simulink model "MrasObserver"  (R2026b)
settings: Solver=VariableStepAuto
undefined symbols (not defined in the file or in its folder): mras_parameters
settings Model: Creator=24322  LastModifiedBy=24322

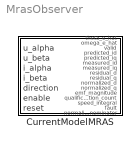
== system MrasObserver ==
  CurrentModelMRAS : Subsystem  mask{cfg=mras_parameters()}
      mask prompts: cfg "MRAS configuration"

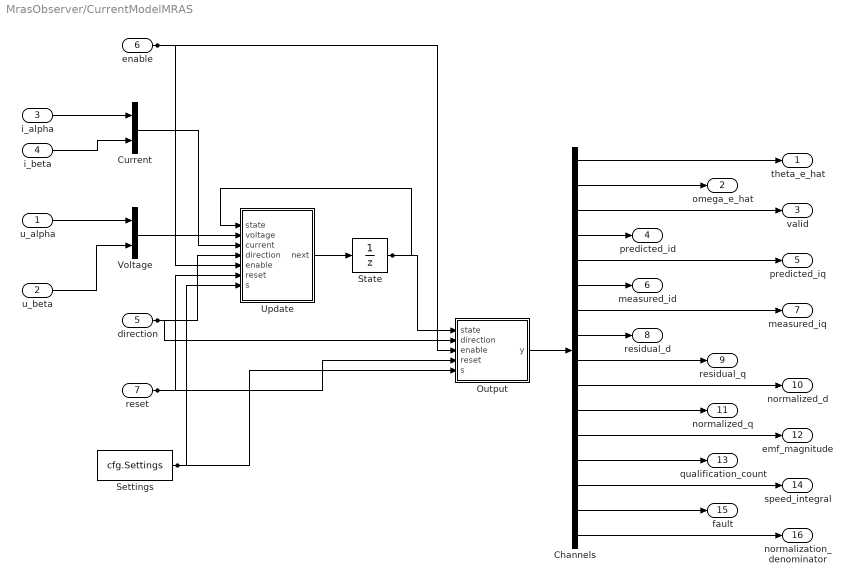
== system MrasObserver/CurrentModelMRAS ==
  u_alpha : Inport  SampleTime=cfg.Ts
  u_beta : Inport  Port=2  SampleTime=cfg.Ts
  i_alpha : Inport  Port=3  SampleTime=cfg.Ts
  i_beta : Inport  Port=4  SampleTime=cfg.Ts
  direction : Inport  Port=5  SampleTime=cfg.Ts
  enable : Inport  Port=6  SampleTime=cfg.Ts
  reset : Inport  Port=7  SampleTime=cfg.Ts
  Channels : Demux  Outputs=16
  Current : Mux  Inputs=2
  Output : MATLAB Function  TreatAsAtomicUnit=on
  Settings : Constant  Value=cfg.Settings
  State : UnitDelay  InitialCondition=zeros(21,1)  SampleTime=cfg.Ts
  Update : MATLAB Function  TreatAsAtomicUnit=on
  Voltage : Mux  Inputs=2
  theta_e_hat : Outport
  omega_e_hat : Outport  Port=2
  valid : Outport  Port=3
  predicted_id : Outport  Port=4
  predicted_iq : Outport  Port=5
  measured_id : Outport  Port=6
  measured_iq : Outport  Port=7
  residual_d : Outport  Port=8
  residual_q : Outport  Port=9
  normalized_d : Outport  Port=10
  normalized_q : Outport  Port=11
  emf_magnitude : Outport  Port=12
  qualification_count : Outport  Port=13
  speed_integral : Outport  Port=14
  fault : Outport  Port=15
  normalization_denominator : Outport  Port=16
  wires:
  Channels/16 -> normalization_denominator/1
  Channels/15 -> fault/1
  Channels/14 -> speed_integral/1
  Channels/13 -> qualification_count/1
  Channels/12 -> emf_magnitude/1
  Channels/11 -> normalized_q/1
  Channels/10 -> normalized_d/1
  Channels/9 -> residual_q/1
  Channels/8 -> residual_d/1
  Channels/7 -> measured_iq/1
  Channels/6 -> measured_id/1
  Channels/5 -> predicted_iq/1
  Channels/4 -> predicted_id/1
  Channels/3 -> valid/1
  Channels/2 -> omega_e_hat/1
  Channels/1 -> theta_e_hat/1
  Output/1(y) -> Channels/1
  Update/1(next) -> State/1
  Settings/1 -> Update/7(s), Output/5(s)
  reset/1 -> Update/6(reset), Output/4(reset)
  enable/1 -> Update/5(enable), Output/3(enable)
  direction/1 -> Update/4(direction), Output/2(direction)
  Current/1 -> Update/3(current)
  Voltage/1 -> Update/2(voltage)
  State/1 -> Update/1(state), Output/1(state)
  i_beta/1 -> Current/2
  i_alpha/1 -> Current/1
  u_beta/1 -> Voltage/2
  u_alpha/1 -> Voltage/1

== matlab function MrasObserver/CurrentModelMRAS/Output ==
  data: state input; y output; direction input; enable input; reset input; s input
function y=mras_output(state,direction,enable,reset,s)
%MRAS_OUTPUT State-only observer outputs; voltage is consumed by next-state only.
% Diagnostics describe the previous processed measurement (one Ts old).
%#codegen
y=zeros(16,1,'like',state);
if ~all(isfinite(s)) || s(1)<=0 || s(3)<=0 || s(4)<=0 || ...
        ~isfinite(enable) || ~isfinite(reset) || ~isfinite(direction) || ...
        (direction~=0 && abs(direction)~=1)
    y(15)=2;return;
end
y(1)=s(9);
if enable<.5 || reset>.5 || direction==0 || direction~=state(12),return;end
y(1)=state(1);y(2)=state(3);
y(3)=double(state(11)>=s(17) && state(20)==0);
y(4:5)=state(13:14);y(6:7)=state(4:5);y(8:9)=state(15:16);
y(10:11)=state(17:18);y(12)=state(19);y(13)=state(11);
y(14)=state(2);y(15)=state(20);y(16)=state(21);
end

== matlab function MrasObserver/CurrentModelMRAS/Update ==
  data: state input; next output; voltage input; current input; direction input; enable input; reset input; s input
function next=mras_step(state,voltage,current,direction,enable,reset,s)
%MRAS_STEP One-step measured-current model and PI speed adaptation (SPMSM).
% State and settings indices are documented in parameter/README.md.
% No integrated current estimate replaces the previous measured dq current.
%#codegen
next=state;
if isfinite(enable) && isfinite(reset) && (enable<.5 || reset>.5)
    next=zeros(21,1,'like',state);next(1)=s(9);return;
end
if ~all(isfinite(s)) || s(1)<=0 || s(3)<=0 || s(4)<=0 || ...
        ~isfinite(enable) || ~isfinite(reset) || ~isfinite(direction) || ...
        (direction~=0 && abs(direction)~=1)
    next=zeros(21,1,'like',state);next(20)=2;return;
end
if direction==0
    next=zeros(21,1,'like',state);next(1)=s(9);return;
end
if state(20)>0,next(11)=0;next(3)=0;return;end
if ~all(isfinite(voltage)) || ~all(isfinite(current))
    next(20)=1;next(11)=0;next(3)=0;return;
end
if state(12)~=direction
    next=zeros(21,1,'like',state);next(1)=s(9);
    next(2)=direction*s(10);next(3)=direction*s(10);next(12)=direction;return;
end
ts=s(1);resistance=s(2);inductance=s(3);flux=s(4);
theta=state(1);cosine=cos(theta);sine=sin(theta);
measured=[cosine*current(1)+sine*current(2);-sine*current(1)+cosine*current(2)];
applied=[cosine*voltage(1)+sine*voltage(2);-sine*voltage(1)+cosine*voltage(2)];
omega=state(3);integral=state(2);count=cast(0,'like',state);
if state(8)>.5
    previous=state(4:5);previousVoltage=state(6:7);
    predicted=previous+(ts/inductance)*(previousVoltage-resistance*previous+ ...
        omega*inductance*[previous(2);-previous(1)]-[0;omega*flux]);
    residual=measured-predicted;
    filtered=state(9:10)+s(8)*(residual-state(9:10));
    denominator=ts*omega*flux/inductance;
    floorValue=ts*s(11)*flux/inductance;
    denominator=direction*max(abs(denominator),floorValue);
    normalizedD=filtered(1)/denominator;normalizedQ=filtered(2)/denominator;
    error=min(max(normalizedD,-1),1);
    unlimited=integral+s(5)*error;
    omega=direction*min(max(direction*unlimited,s(11)),s(12));
    integral=integral+ts*(s(6)*error+s(7)*(omega-unlimited));
    integral=min(max(integral,-s(12)),s(12));
    emf=[0;state(3)*flux]-(inductance/ts)*filtered;
    magnitude=hypot(emf(1),emf(2));
    qualified=abs(omega)>=s(13) && magnitude>=s(14) && ...
        abs(normalizedD)<=s(15) && abs(normalizedQ)<=s(16);
    if qualified,count=min(state(11)+1,s(17));end
    next(9:10)=filtered;next(13:14)=predicted;next(15:16)=residual;
    next(17)=normalizedD;next(18)=normalizedQ;next(19)=magnitude;next(21)=denominator;
end
next(1)=atan2(sin(theta+ts*omega),cos(theta+ts*omega));
next(2)=integral;next(3)=omega;next(4:5)=measured;next(6:7)=applied;
next(8)=1;next(11)=count;next(12)=direction;
end
